simulink model "q_aero_2dof_lqr_control_dup"  (R2025a)
settings: Solver=ode1  StartTime=0.0  StopTime=30  FixedStep=0.002  RelTol=1e-3  EnableMultiTasking=on
PreLoadFcn:
  | quanser_aero_lqr
undefined symbols (not defined in the file or in its folder): K
libraries: simulink_extras x4, quarc_library x3
settings Model: SimulationMode=external  ExtModeTrigDuration=15000  Creator=MLevis  LastModifiedBy=e82540u
settings SolverCC: AlgebraicLoopSolver=TrustRegion  PositivePriorityOrder=on
settings DataIOCC: LimitDataPoints=on  SaveFormat=Array  ReturnWorkspaceOutputs=off
settings DebuggingCC: SolverPrmCheckMsg=warning  UnconnectedInputMsg=warning  UnconnectedOutputMsg=warning  UnconnectedLineMsg=warning  SFUnexpectedBacktrackingDiag=warning  SFNoUnconditionalDefaultTransitionDiag=warning  SFExecutionAtInitializationDiag=none  ArithmeticOperatorsInVariantConditions=warning
settings ModelReferenceCC: PropagateSignalLabelsOutOfModel=off
settings SFSimCC: SimUseLocalCustomCode=off  CustomCodeUndefinedFunction=UseInterfaceOnly
settings RTWCC: SystemTargetFile=quarc_win64.tlc  TemplateMakefile=quarc_default_tmf  RTWUseLocalCustomCode=off  Toolchain=QUARC win64 | nmake (64-bit Windows)  BuildConfiguration=Faster Runs  GPUComputeCapability=3.5  Description=QUARC Win64 Target Using Toolchain
settings CodeAppCC: StateflowObjectComments=on
settings STFCustomTargetCC: SystemTargetFile=quarc_win64.tlc  MultiwordLength=2048.0  DynamicStringBufferSize=256.0  ConcurrentExecutionCompliant=on  UseToolchainInfoCompliant=on
settings GRTTargetCC: ExtMode=on  ExtModeMexFile=quarc_comm  TargetLangStandard=C89/C90 (ANSI)  ParMdlRefBuildCompliant=off  CompOptLevelCompliant=off  CombineOutputUpdateFcns=off  MatFileLogging=off  CPPClassGenCompliant=off  GRTInterface=on
settings ConfigComp: CovMetricSettings=dw  CovSaveCumulativeToWorkspaceVar=on  CovSaveSingleToWorkspaceVar=on  CovExternalEMLEnable=off  CovSFcnEnable=off

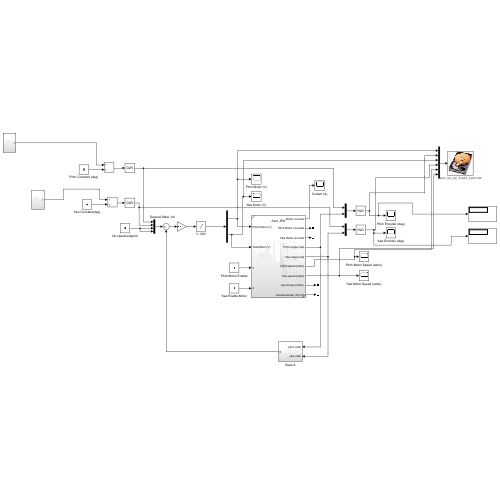
[thumbnail: Simulink's stored preview of the top-level diagram]
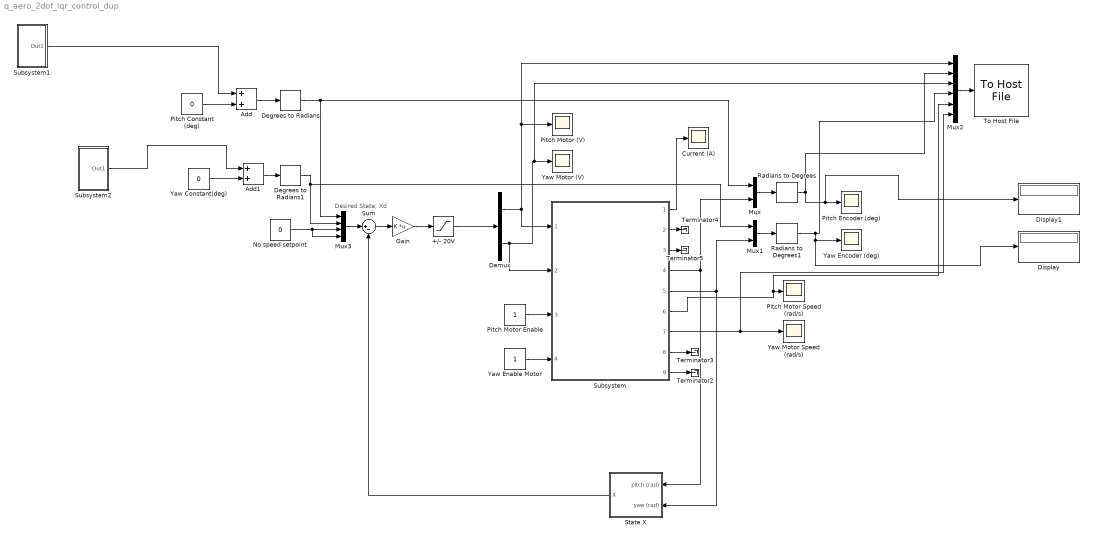
== system q_aero_2dof_lqr_control_dup ==
  note: Desired State; Xd
  +/- 20V : Saturate  UpperLimit=20  LowerLimit=-20
  Add : Sum
  Add1 : Sum
  Current (A) : Scope
      settings: TimeSpan=5  ActiveDisplayYMinimum=-3.2333994870542253  ActiveDisplayYMaximum=2.9682065217391305  DataLoggingSaveFormat=Array
  Degrees to Radians : simulink_extras/Transformations/Degrees to Radians
  Degrees to Radians1 : simulink_extras/Transformations/Degrees to Radians
  Demux : Demux  Outputs=2
  Display : Display
  Display1 : Display
  Gain : Gain  Gain=K  Multiplication=Matrix(K*u)
  Mux : Mux  Inputs=2
  Mux1 : Mux  Inputs=2
  Mux2 : Mux  Inputs=6
  Mux3 : Mux
  No speed setpoint : Constant  Value=0
  Pitch Constant (deg) : Constant  Value=0
  Pitch Encoder (deg) : Scope
      settings: TimeSpan=30  ActiveDisplayYMinimum=-38.26340620212148  ActiveDisplayYMaximum=22.652136380460348  DataLoggingMaxPoints=15000  DataLoggingVariableName=ScopeData3  DataLoggingSaveFormat=Array
  Pitch Motor (V) : Scope
      settings: TimeSpan=30  ActiveDisplayYMinimum=-58.872834942848577  ActiveDisplayYMaximum=54.772752938314753  DataLoggingMaxPoints=15000  DataLoggingVariableName=ScopeData2  DataLoggingSaveFormat=Array
  Pitch Motor Enable : Constant
  Pitch Motor Speed (rad/s) : Scope
      settings: TimeSpan=10  ActiveDisplayYMinimum=-1000  ActiveDisplayYMaximum=1000  DataLoggingSaveFormat=Array
  Radians to Degrees : simulink_extras/Transformations/Radians to Degrees
  Radians to Degrees1 : simulink_extras/Transformations/Radians to Degrees
  State X : Subsystem
  Subsystem : Subsystem  ReferencedSubsystem=Aero_RW
  Subsystem1 : Subsystem
  Subsystem2 : Subsystem
  Sum : Sum  Inputs=|+-
  Terminator{2..5} (4 alike) : Terminator
  To Host File : quarc_library/Sinks/To Host/To Host File  source=Specify via dialog (do not evaluate)  file_name=aero_lqr_rsp_fixed2_sys4.mat  variable_name=lqr_rsp  decimation=1  sample_time=-1  file_format=MAT-file v.4  options=No header or footer  append=off  final_file_name=aero_lqr_rsp_fixed2_sys4.mat  encoding=Default  bitrate=0
  Yaw Constant(deg) : Constant  Value=0
  Yaw Enable Motor : Constant
  Yaw Encoder (deg) : Scope
      settings: TimeSpan=30  ActiveDisplayYMinimum=-120  ActiveDisplayYMaximum=120  DataLoggingMaxPoints=15000  DataLoggingVariableName=ScopeData4  DataLoggingSaveFormat=Array
  Yaw Motor (V) : Scope
      settings: TimeSpan=30  ActiveDisplayYMinimum=-41.025670028136645  ActiveDisplayYMaximum=53.25678708802522  DataLoggingMaxPoints=15000  DataLoggingVariableName=ScopeData5  DataLoggingSaveFormat=Array
  Yaw Motor Speed (rad/s) : Scope
      settings: TimeSpan=10  ActiveDisplayYMinimum=-100000  ActiveDisplayYMaximum=100000  DataLoggingVariableName=ScopeData8  DataLoggingSaveFormat=Array
  wires:
  Degrees to Radians/1 -> Mux3/1, Mux/1
  Degrees to Radians1/1 -> Mux3/2, Mux1/1
  Pitch Constant (deg)/1 -> Add/2
  Add/1 -> Degrees to Radians/1
  Yaw Constant(deg)/1 -> Add1/2
  Add1/1 -> Degrees to Radians1/1
  Mux/1 -> Radians to Degrees/1
  Radians to Degrees/1 -> Mux2/2, Display1/1, Pitch Encoder (deg)/1
  Radians to Degrees1/1 -> Yaw Encoder (deg)/1, Display/1, Mux2/4
  Pitch Motor Enable/1 -> Subsystem/3
  Yaw Enable Motor/1 -> Subsystem/4
  Gain/1 -> +/- 20V/1
  Demux/1 -> Subsystem/1, Mux2/1, Pitch Motor (V)/1
  Demux/2 -> Mux2/3, Yaw Motor (V)/1, Subsystem/2
  Sum/1 -> Gain/1
  Mux1/1 -> Radians to Degrees1/1
  Mux3/1 -> Sum/1
  No speed setpoint/1 -> Mux3/4, Mux3/3
  +/- 20V/1 -> Demux/1
  State X/1(X) -> Sum/2
  Subsystem/4 -> Mux/2, State X/1(pitch (rad))
  Subsystem/5 -> Mux1/2, State X/2(yaw (rad))
  Mux2/1 -> To Host File/1
  Subsystem/9 -> Terminator2/1
  Subsystem/8 -> Terminator3/1
  Subsystem/6 -> Mux2/5, Pitch Motor Speed (rad/s)/1
  Subsystem/7 -> Mux2/6, Yaw Motor Speed (rad/s)/1
  Subsystem/1 -> Current (A)/1
  Subsystem/3 -> Terminator5/1
  Subsystem/2 -> Terminator4/1
  Subsystem2/1(Out1) -> Add1/1
  Subsystem1/1(Out1) -> Add/1

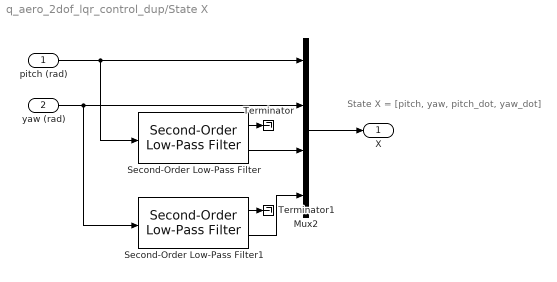
== system q_aero_2dof_lqr_control_dup/State X ==
  note: State X = [pitch, yaw, pitch_dot, yaw_dot]
  pitch (rad) : Inport
  yaw (rad) : Inport  Port=2
  Mux2 : Mux
  "Second-Order Low-Pass Filter " : quarc_library/Continuous/Second-Order Low-Pass Filter  params_source=Internal (dialog parameters)  input_width=50  input_zeta=0.8  input_init=0
  "Second-Order Low-Pass Filter1 " : quarc_library/Continuous/Second-Order Low-Pass Filter  params_source=Internal (dialog parameters)  input_width=50  input_zeta=0.8  input_init=0
  Terminator : Terminator
  Terminator1 : Terminator
  X : Outport
  wires:
  Mux2/1 -> X/1
  yaw (rad)/1 -> "Second-Order Low-Pass Filter1 "/1, Mux2/2
  pitch (rad)/1 -> "Second-Order Low-Pass Filter "/1, Mux2/1
  "Second-Order Low-Pass Filter "/2 -> Mux2/3
  "Second-Order Low-Pass Filter1 "/2 -> Mux2/4
  "Second-Order Low-Pass Filter "/1 -> Terminator/1
  "Second-Order Low-Pass Filter1 "/1 -> Terminator1/1

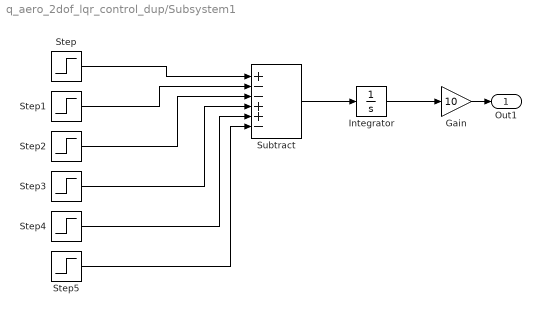
== system q_aero_2dof_lqr_control_dup/Subsystem1 ==
  Gain : Gain  Gain=10
  Integrator : Integrator
  Step : Step  After=2  SampleTime=5
  Step1 : Step  After=2  SampleTime=6
  Step2 : Step  After=2  SampleTime=10
  Step3 : Step  After=2  SampleTime=12
  Step4 : Step  After=2  SampleTime=15
  Step5 : Step  After=2  SampleTime=17
  Subtract : Sum  Inputs=+--++-
  Out1 : Outport
  wires:
  Gain/1 -> Out1/1
  Step3/1 -> Subtract/4
  Step/1 -> Subtract/1
  Subtract/1 -> Integrator/1
  Step4/1 -> Subtract/5
  Step5/1 -> Subtract/6
  Integrator/1 -> Gain/1
  Step1/1 -> Subtract/2
  Step2/1 -> Subtract/3

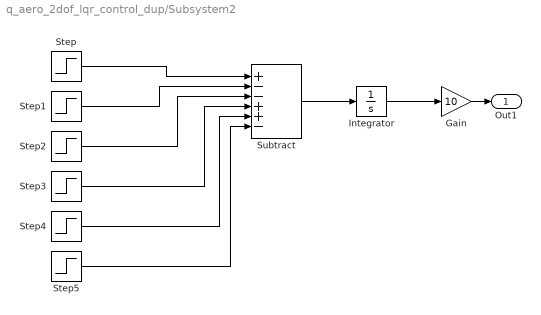
== system q_aero_2dof_lqr_control_dup/Subsystem2 ==
  Gain : Gain  Gain=10
  Integrator : Integrator
  Step : Step  After=2  SampleTime=12.5
  Step1 : Step  After=2  SampleTime=13.5
  Step2 : Step  After=2  SampleTime=25
  Step3 : Step  After=2  SampleTime=27
  Step4 : Step  After=2  SampleTime=47.5
  Step5 : Step  After=2  SampleTime=49.5
  Subtract : Sum  Inputs=+--++-
  Out1 : Outport
  wires:
  Gain/1 -> Out1/1
  Step3/1 -> Subtract/4
  Step/1 -> Subtract/1
  Subtract/1 -> Integrator/1
  Step4/1 -> Subtract/5
  Step5/1 -> Subtract/6
  Integrator/1 -> Gain/1
  Step1/1 -> Subtract/2
  Step2/1 -> Subtract/3
